simulink model "MC710_ID2"  (Simulink 7.2)
settings: Solver=FixedStepDiscrete  StartTime=0.0  StopTime=5  FixedStep=0.0005  RelTol=1e-3
undefined symbols (not defined in the file or in its folder): QEIInit, sendPOS, y1
libraries: dsPICdrivers x9, simulink x5
settings Model: Creator=ASL_Lab  LastModifiedBy=magicNTU
settings OptimizationCC: InlineParams=on  InlineInvariantSignals=on  InitFltsAndDblsToZero=on  OptimizeModelRefInitCode=on  LifeSpan=1
settings DebuggingCC: SaveWithParameterizedLinksMsg=none  MultiTaskDSMMsg=none  MultiTaskCondExecSysMsg=warning
settings HardwareCC: ProdBitPerInt=16  ProdEndianess=LittleEndian  ProdWordSize=16  ProdHWDeviceType=16-bit Generic
settings RTWCC: SystemTargetFile=dspic.tlc  TemplateMakefile=dspic_pic30_gcc.tmf  PostCodeGenCommand=dsPIC_Compile()  Description=Embedded Target for Microchip dsPIC (real-time)  GenerateReport=on  ProcessScript=dspic_make_rtw_hook  CustomSource=QEI_ID2.c  IncludeHyperlinkInReport=on  LaunchReport=on  GenerateTraceInfo=on  GenerateTraceReport=on  GenerateTraceReportSl=on  GenerateTraceReportSf=on  GenerateTraceReportEml=on
settings CodeAppCC: IgnoreCustomStorageClasses=off
settings STFCustomTargetCC: ModelReferenceCompliant=off  IncludeMdlTerminateFcn=off  CombineOutputUpdateFcns=on  SuppressErrorStatus=on  ERTCustomFileBanners=on  SupportContinuousTime=off  SupportNonInlinedSFcns=off  SystemTargetFile=dspic.tlc
settings ERTTargetCC: MultiwordLength=2048  ModelReferenceCompliant=off  CompOptLevelCompliant=off  IncludeMdlTerminateFcn=off  SuppressErrorStatus=on  ERTFirstTimeCompliant=off  ModelStepFunctionPrototypeControlCompliant=off  CPPClassGenCompliant=off  ExtModeMexFile=noextcomm  InlinedParameterPlacement=NonHierarchical  ERTSrcFileBannerTemplate=dsPIC_code_template.cgt  ERTHdrFileBannerTemplate=dsPIC_code_template.cgt  ERTDataSrcFileTemplate=dsPIC_code_template.cgt  ERTDataHdrFileTemplate=dsPIC_code_template.cgt  ERTCustomFileTemplate=dsPIC_main.tlc
settings CustomProperty: DataType=string  Value=C:\PROGRA~1\MATLAB\R2008b\bin\win32\gmake

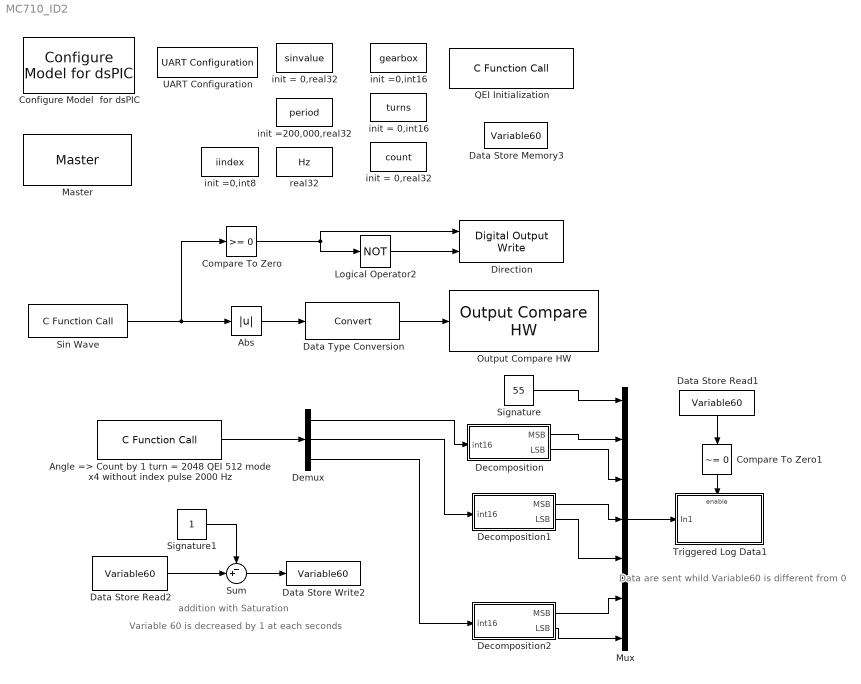
== system MC710_ID2 ==
  note: Variable 60 is decreased by 1 at each seconds
  note: addition
      | with Saturation
  note: Data are sent whild Variable60 is different from 0
  Abs : Abs  OutDataType=sfix(16)  OutScaling=2^0
  Angle => Count by 1 turn = 2048 QEI 512 mode x4 without index pulse 2000 Hz : dsPICdrivers/OTHERS/C Function Call  Tag=dsPIC_dsPIC_CFunctionCall  fctName='sendPOS'  INPUT_SIZE=1  INPUT1=--  INPUT2=--  INPUT3=--  OUTPUT_SIZE=3  OUTPUT1=int16  SampleTime=.0005  InputType=[ ]  OutputType=[ 3 ]  FctDeclaration=extern void sendPOS(int16_T* y1);  FctCall=sendPOS(*%y1);  OrderingInOutPopup=None
  Compare To Zero : simulink/Logic and Bit Operations/Compare To Zero  SystemSampleTime=-1  relop=>=  LogicOutDataTypeMode=boolean  ZeroCross=off
  Compare To Zero1 : simulink/Logic and Bit Operations/Compare To Zero  Orientation=down  SystemSampleTime=-1  relop=~=  LogicOutDataTypeMode=boolean  ZeroCross=off
  Configure Model  for dsPIC : dsPICdrivers/Simulink Configuration/Configure Model  for dsPIC
  Data Store Memory3 : DataStoreMemory  DataStoreName=Variable60  ReadBeforeWriteMsg=warning  WriteAfterWriteMsg=warning  WriteAfterReadMsg=warning  InitialValue=1  DataType=uint8  OutDataType=sfix(16)  OutScaling=2^0  OutDataTypeStr=uint8
  Data Store Read1 : DataStoreRead  Orientation=down  DataStoreName=Variable60  SampleTime=0.1
  Data Store Read2 : DataStoreRead  DataStoreName=Variable60  SampleTime=0.1
  Data Store Write2 : DataStoreWrite  DataStoreName=Variable60  SampleTime=.1
  Data Type Conversion : DataTypeConversion  OutDataType=sfix(16)  OutScaling=2^0  RndMeth=Nearest
  Decomposition : Subsystem
  Decomposition1 : Subsystem
  Decomposition2 : Subsystem
  Demux : Demux  Outputs=3
  Direction : dsPICdrivers/Digital I//O/Digital Output Write  Tag=dsPIC_Digital_Output  Priority=5  PORT=F  Pin=[2 3]  Simultaneous=off  OrderingInOutPopup=None
  Logical Operator2 : Logic  Operator=NOT  Inputs=1  OutDataTypeMode=boolean  OutDataTypeStr=boolean
  Master : dsPICdrivers/Master  Tag=dsPIC_MASTER  TimeStepType=Timer1  picType=33fJ256MC710  fcy=36800000  Quartz_33f=20e6  PLLActive_33f=on  fcyDesired_33f=36800000  tmr1="[1  18399  0]"  tmr1Info="Time Step : 0.0005  ;   Error : 0%  PR1=18399"  tmr2345="[1  0  0  0  0  0  0  0]"  tmr2345cfg=[-1 -1 -1 -1 -1 -1 -1 -1]  IOautoConf=on  typePort="[ 0   0   0   0   0   0   0   0   0   0   0   0   0   0   0   0   0   0   0   0   0   0   0   0   0   0   0   0   0   0   0   0   0   0   0   0   0   0   0   0   0   0   0   0   0   0   0   0   0  24   0   0   0   0   0   0   0   0   0   0   0   0   0   0   0   0   0   0   0   0   0   0   0   0   0   0   0   0   0   0   0   0  10  10   4   5   0   0   0   0   0   0   0   0   0   0   0   0   0   0   0   0   0   0   0   0   0   0   0   0   0   0 ]"  TRIS="[ 65535  65535  65535  65533  65535  65523  65535 ]"  ADPCFG=0  MasterBusyPort=None  MasterOverloadPort=None  FOSC=Quartz (XT - HS)  ClockSwitchMonitor=Both disabled  TempProtection_33f=TEMP_ON  FPBOR=<empty>  PWRT=64ms  MCLR=<empty>  PowerSave=off  OverrideFcy=off  NewFcy=1e6  PR2345="[1839  65535  65535  65535  65535  65535  65535  65535]"
  Mux : Mux  Inputs=7
  Output Compare HW : dsPICdrivers/Peripheral I//O/Output Compare HW  Tag=dsPIC_OC_HW_out  Priority=5  OC_Mode=PWM duty cycle (robust)  Timer=2  CHANNEL=[2]  Channel_UP_Down_Periode=[5]  PeriodeInput=off  MaxChannel=5e-005  MaxName=' OCmax '  Precision=[10.8455]  Status=OK  SafeMarge=[0]  PortLetter=[68]  PortNumber=[1]  MaxValues=[1839]  NPORTS=1
  QEI Initialization : dsPICdrivers/OTHERS/C Function Call  Tag=dsPIC_dsPIC_CFunctionCall  fctName='QEIInit'  INPUT_SIZE=1  INPUT1=--  INPUT2=--  INPUT3=--  OUTPUT_SIZE=1  OUTPUT1=--  SampleTime=inf  InputType=[ ]  OutputType=[ ]  FctDeclaration=extern void QEIInit();  FctCall=QEIInit();  OrderingInOutPopup=None
  Signature : Constant  Value=55  OutDataTypeMode=uint8  OutDataType=sfix(16)  OutScaling=2^0  OutDataTypeStr=uint8
  Signature1 : Constant  OutDataTypeMode=uint8  OutDataType=sfix(16)  OutScaling=2^0  OutDataTypeStr=uint8
  Sin Wave : dsPICdrivers/OTHERS/C Function Call  Tag=dsPIC_dsPIC_CFunctionCall  fctName='sinout'  INPUT_SIZE=1  INPUT1=--  INPUT2=--  INPUT3=--  OUTPUT_SIZE=1  OUTPUT1=real32  SampleTime=.0005  InputType=[ ]  OutputType=[ 7 ]  FctDeclaration=extern real32_T sinout();  FctCall=%y1 = sinout();  OrderingInOutPopup=None
  Sum : Sum  Inputs=-+|  AccumDataTypeStr=uint16  OutDataTypeMode=uint8  OutDataType=sfix(16)  OutScaling=2^0  OutDataTypeStr=uint8  SampleTime=.1  SaturateOnIntegerOverflow=on
  Triggered Log Data1 : Subsystem
  UART Configuration : dsPICdrivers/Serial PORT/UART Configuration  Tag=dsPIC_config_UART  UART=2  proposed_BAUD=115200  ALT_TX_RX=off  InterruptTxWhen=When Transmit Buffer is empty  TXInterruptPri=7  TxBufferSize=32  TXEN=on  InterruptRxWhen=When Receive Buffer is full (contain 4 characters)  RXInterruptPri=1  RxBufferSize=4  BAUD=115200  UxBRG=19  Info="UxBRG = 19   ||  Real Baud : 115000   ||  % error : -0.17361  ||  max 5.75 Bytes / Step"  RealBaud=0
  init = 0,int16 : DataStoreMemory  DataStoreName=turns  ReadBeforeWriteMsg=warning  WriteAfterWriteMsg=warning  WriteAfterReadMsg=warning  DataType=int16  OutDataType=sfix(16)  OutScaling=2^0  OutDataTypeStr=int16
      settings: RTWStateStorageClass=ExportedGlobal
  init = 0,real32 : DataStoreMemory  DataStoreName=sinvalue  ReadBeforeWriteMsg=warning  WriteAfterWriteMsg=warning  WriteAfterReadMsg=warning  DataType=single  OutDataType=sfix(16)  OutScaling=2^0  OutDataTypeStr=single
      settings: RTWStateStorageClass=ExportedGlobal
  "init = 0,real32 " : DataStoreMemory  DataStoreName=count  ReadBeforeWriteMsg=warning  WriteAfterWriteMsg=warning  WriteAfterReadMsg=warning  DataType=single  OutDataType=sfix(16)  OutScaling=2^0  OutDataTypeStr=single
      settings: RTWStateStorageClass=ExportedGlobal
  init =0,int16 : DataStoreMemory  DataStoreName=gearbox  ReadBeforeWriteMsg=warning  WriteAfterWriteMsg=warning  WriteAfterReadMsg=warning  DataType=int16  OutDataType=sfix(16)  OutScaling=2^0  OutDataTypeStr=int16
      settings: RTWStateStorageClass=ExportedGlobal
  init =0,int8 : DataStoreMemory  DataStoreName=iindex  ReadBeforeWriteMsg=warning  WriteAfterWriteMsg=warning  WriteAfterReadMsg=warning  DataType=int8  OutDataType=sfix(16)  OutScaling=2^0  OutDataTypeStr=int8
      settings: RTWStateStorageClass=ExportedGlobal
  init =200,000,real32 : DataStoreMemory  DataStoreName=period  ReadBeforeWriteMsg=warning  WriteAfterWriteMsg=warning  WriteAfterReadMsg=warning  InitialValue=200000  DataType=single  OutDataType=sfix(16)  OutScaling=2^0  OutDataTypeStr=single
      settings: RTWStateStorageClass=ExportedGlobal
  real32 : DataStoreMemory  DataStoreName=Hz  ReadBeforeWriteMsg=warning  WriteAfterWriteMsg=warning  WriteAfterReadMsg=warning  InitialValue=[.01 .02 .03 .04 .05 .06 .07 .08 .09 .1 .2 .3 .4 .5 .6 .7 .8 .9 1 2]  DataType=single  OutDataType=sfix(16)  OutScaling=2^0  OutDataTypeStr=single
      settings: RTWStateStorageClass=ExportedGlobal
  wires:
  Data Type Conversion/1 -> Output Compare HW/1
  Abs/1 -> Data Type Conversion/1
  Logical Operator2/1 -> Direction/2
  Demux/1 -> Decomposition/1(int16)
  Angle => Count by 1 turn = 2048 QEI 512 mode x4 without index pulse 2000 Hz/1 -> Demux/1
  Demux/2 -> Decomposition1/1(int16)
  Demux/3 -> Decomposition2/1(int16)
  Sin Wave/1 -> Abs/1, Compare To Zero/1
  Compare To Zero/1 -> Logical Operator2/1, Direction/1
  Data Store Read2/1 -> Sum/2
  Signature1/1 -> Sum/1
  Sum/1 -> Data Store Write2/1
  Signature/1 -> Mux/1
  Decomposition/2(LSB) -> Mux/3
  Decomposition1/1(MSB) -> Mux/4
  Decomposition2/1(MSB) -> Mux/6
  Decomposition2/2(LSB) -> Mux/7
  Mux/1 -> Triggered Log Data1/1(In1)
  Compare To Zero1/1 -> Triggered Log Data1/Enable
  Data Store Read1/1 -> Compare To Zero1/1
  Decomposition1/2(LSB) -> Mux/5
  Decomposition/1(MSB) -> Mux/2

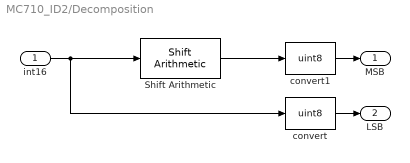
== system MC710_ID2/Decomposition ==
  int16 : Inport
  Shift Arithmetic : simulink/Logic and Bit Operations/Shift Arithmetic  SystemSampleTime=-1  nBitShiftRight=8  nBinPtShiftRight=0
  convert : DataTypeConversion  OutDataTypeMode=uint8  OutDataType=sfix(16)  OutScaling=2^0  OutDataTypeStr=uint8  ConvertRealWorld=Stored Integer (SI)
  convert1 : DataTypeConversion  OutDataTypeMode=uint8  OutDataType=sfix(16)  OutScaling=2^0  OutDataTypeStr=uint8  ConvertRealWorld=Stored Integer (SI)
  MSB : Outport
  LSB : Outport  Port=2
  wires:
  int16/1 -> convert/1, Shift Arithmetic/1
  Shift Arithmetic/1 -> convert1/1
  convert1/1 -> MSB/1
  convert/1 -> LSB/1

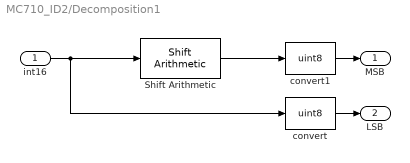
== system MC710_ID2/Decomposition1 ==
  int16 : Inport
  Shift Arithmetic : simulink/Logic and Bit Operations/Shift Arithmetic  SystemSampleTime=-1  nBitShiftRight=8  nBinPtShiftRight=0
  convert : DataTypeConversion  OutDataTypeMode=uint8  OutDataType=sfix(16)  OutScaling=2^0  OutDataTypeStr=uint8  ConvertRealWorld=Stored Integer (SI)
  convert1 : DataTypeConversion  OutDataTypeMode=uint8  OutDataType=sfix(16)  OutScaling=2^0  OutDataTypeStr=uint8  ConvertRealWorld=Stored Integer (SI)
  MSB : Outport
  LSB : Outport  Port=2
  wires:
  convert/1 -> LSB/1
  convert1/1 -> MSB/1
  Shift Arithmetic/1 -> convert1/1
  int16/1 -> Shift Arithmetic/1, convert/1

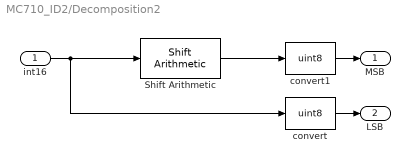
== system MC710_ID2/Decomposition2 ==
  int16 : Inport
  Shift Arithmetic : simulink/Logic and Bit Operations/Shift Arithmetic  SystemSampleTime=-1  nBitShiftRight=8  nBinPtShiftRight=0
  convert : DataTypeConversion  OutDataTypeMode=uint8  OutDataType=sfix(16)  OutScaling=2^0  OutDataTypeStr=uint8  ConvertRealWorld=Stored Integer (SI)
  convert1 : DataTypeConversion  OutDataTypeMode=uint8  OutDataType=sfix(16)  OutScaling=2^0  OutDataTypeStr=uint8  ConvertRealWorld=Stored Integer (SI)
  MSB : Outport
  LSB : Outport  Port=2
  wires:
  int16/1 -> convert/1, Shift Arithmetic/1
  Shift Arithmetic/1 -> convert1/1
  convert1/1 -> MSB/1
  convert/1 -> LSB/1

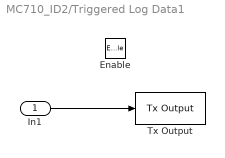
== system MC710_ID2/Triggered Log Data1 ==
  In1 : Inport
  Enable : EnablePort
  Tx Output : dsPICdrivers/Serial PORT/Tx Output  Tag=dsPIC_TX  Priority=5  UART=2  OrderingInOutPopup=None
  wires:
  In1/1 -> Tx Output/1
